simulink library "Motor_Lib"  (R2025a)
settings: Solver=ode45  StartTime=0.0  StopTime=10.0  RelTol=1e-3  EnableMultiTasking=on
libraries: fl_lib x44, ee_lib x1, $bdroot x1, sdl_lib x1
Description:
  | Copyright 2015-2025 The MathWorks, Inc.
settings Model: Creator=smiller  LastModifiedBy=smiller
settings SolverCC: AlgebraicLoopSolver=TrustRegion
settings DataIOCC: LimitDataPoints=on  SaveFormat=Array  ReturnWorkspaceOutputs=off
settings OptimizationCC: ReuseModelBlockBuffer=off  ExpressionDepthLimit=2147483647.0  LifeSpan=inf
settings DebuggingCC: UnderspecifiedInitializationDetection=Classic  MergeDetectMultiDrivingBlocksExec=none  SolverPrmCheckMsg=warning  UnconnectedInputMsg=warning  UnconnectedOutputMsg=warning  UnconnectedLineMsg=warning  AllowSymbolicDim=off  StateNameClashWarn=warning  PregeneratedLibrarySubsystemCodeDiagnostic=none  SFUnexpectedBacktrackingDiag=warning  SFNoUnconditionalDefaultTransitionDiag=warning  SFExecutionAtInitializationDiag=none  ArithmeticOperatorsInVariantConditions=warning
settings HardwareCC: ProdBitPerPointer=32.0  ProdBitPerSizeT=32.0  ProdBitPerPtrDiffT=32.0  ProdLargestAtomicFloat=None  ProdIntDivRoundTo=Undefined  ProdEndianess=Unspecified  ProdWordSize=32.0  ProdHWDeviceType=32-bit Generic
settings ModelReferenceCC: EnableRefExpFcnMdlSchedulingChecks=on  PropagateSignalLabelsOutOfModel=off
settings SFSimCC: SimUseLocalCustomCode=off  CustomCodeUndefinedFunction=UseInterfaceOnly
settings RTWCC: RTWUseLocalCustomCode=off  GPUComputeCapability=3.5  DLArmComputeVersion=19.05
settings CodeAppCC: StateflowObjectComments=on
settings GRTTargetCC: TargetLangStandard=C89/C90 (ANSI)
settings ConfigComp: CovMetricSettings=dw  CovSaveCumulativeToWorkspaceVar=on  CovSaveSingleToWorkspaceVar=on  CovExternalEMLEnable=off  CovSFcnEnable=off

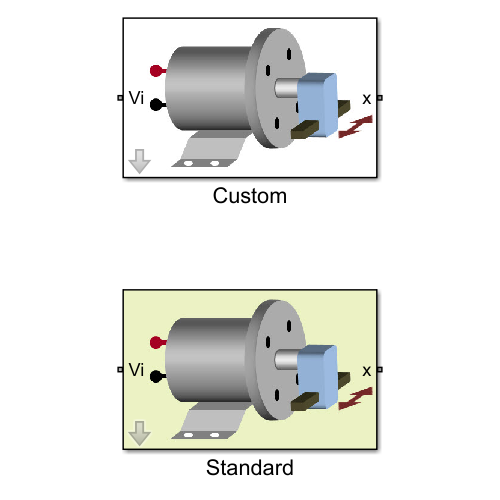
[thumbnail: Simulink's stored preview of the top-level diagram]
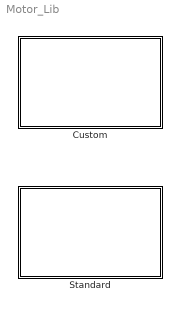
== system Motor_Lib ==
  Custom : Subsystem  mask(Servo and controller){G=0.5e-3/(pi/2), x_max=0.5, J=1e-4, lambda=0.01, R=10, L=2.5, Kt=0.04, R_controller=[10e3 10e3 10e3 100e3 50 100e3 10e3]}
      mask prompts: G "Spool travel per rotation (m)"; x_max "Spool travel limit (mm)"; J "Shaft inertia (kg m^2)"; lambda "Shaft damping (Nm/(rad/s))"; R "Winding resistance (ohms)"; L "Winding inductance (H)"; Kt "Torque constant (Nm/A)"; R_controller "[R1 R2 R3 R4 R5 R6 R7] (ohms)"
      mask help: Models a servomotor and controller using Simscape Foundation library components.
      mask DialogControl DescTextVar_copy Prompt: Controller resistance values
      mask Display: image('DC_Motor_Custom_IMAGE.jpg')
  Standard : Subsystem  mask(Servo and controller){G=0.5e-3/(pi/2), x_max=0.5, J=1e-4, lambda=0.01, R=10, L=2.5, Kt=0.04, R_controller=[10e3 10e3 10e3 100e3 50 100e3 10e3]}
      mask prompts: G "Spool travel per rotation (m)"; x_max "Spool travel limit (mm)"; J "Shaft inertia (kg m^2)"; lambda "Shaft damping (Nm/(rad/s))"; R "Winding resistance (ohms)"; L "Winding inductance (H)"; Kt "Torque constant (Nm/A)"; R_controller "[R1 R2 R3 R4 R5 R6 R7] (ohms)"
      mask help: Models a servomotor and controller using Simscape add-on library components.
      mask DialogControl DescTextVar_copy Prompt: Controller resistance values
      mask Display: image('DC_Motor_Standard_IMAGE.jpg')

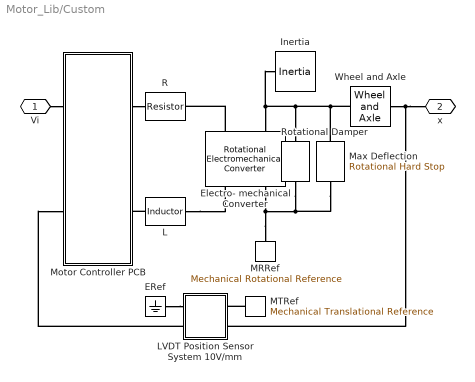
== system Motor_Lib/Custom ==
  ERef : fl_lib/Electrical/Electrical Elements/Electrical Reference
  Electro- mechanical Converter : fl_lib/Electrical/Electrical Elements/Rotational Electromechanical Converter  K=Kt V/(rad/s)  i_specify=off  i_priority=None  i=0 A  i_nominal_specify=off  i_nominal_value=1  i_nominal_unit=A  v_specify=off  v_priority=None  v=0 V  v_nominal_specify=off  v_nominal_value=1  v_nominal_unit=V  t_specify=off  t_priority=None  t=0 N*m  t_nominal_specify=off  t_nominal_value=1  t_nominal_unit=N*m  w_specify=off  w_priority=None  w=0 rad/s  w_nominal_specify=off  w_nominal_value=1  w_nominal_unit=rad/s
  Inertia : fl_lib/Mechanical/Rotational Elements/Inertia  inertia=J kg*m^2  num_ports=foundation.enum.numPorts2.one  w_specify=on  w_priority=High  w=0 rad/s  w_nominal_specify=off  w_nominal_value=1  w_nominal_unit=rad/s  t_specify=off  t_priority=None  t=0 N*m  t_nominal_specify=off  t_nominal_value=1  t_nominal_unit=N*m
  L : fl_lib/Electrical/Electrical Elements/Inductor  l=L H  r=0 Ohm  g=1e-09 1/Ohm  i_specify=off  i_priority=High  i=0 A  i_nominal_specify=off  i_nominal_value=1  i_nominal_unit=A  v_specify=off  v_priority=High  v=0 V  v_nominal_specify=off  v_nominal_value=1  v_nominal_unit=V  i_L_specify=on  i_L_priority=High  i_L=0 A  i_L_nominal_specify=off  i_L_nominal_value=1  i_L_nominal_unit=A
  LVDT Position Sensor System 10V/mm : Subsystem
  MRRef : fl_lib/Mechanical/Rotational Elements/Mechanical Rotational Reference
  MTRef : fl_lib/Mechanical/Translational Elements/Mechanical Translational Reference
  Max Deflection : fl_lib/Mechanical/Rotational Elements/Rotational Hard Stop  upper_bnd=x_max*1e-3/G rad  lower_bnd=-x_max*1e-3/G rad  model=3  stiff_up=1e+06 N*m/rad  stiff_low=1e+06 N*m/rad  D_up=0.05 N*m/(rad/s)  D_low=0.05 N*m/(rad/s)  transition=0.001 rad  coeff_rest=0.7  w_tol=0.1 rad/s  trq_tol=0.001 N*m  w_specify=off  w_priority=None  w=0 rad/s  w_nominal_specify=off  w_nominal_value=1  w_nominal_unit=rad/s  t_specify=off  t_priority=None  t=0 N*m  t_nominal_specify=off  t_nominal_value=1  t_nominal_unit=N*m  phi_specify=on  phi_priority=High  phi=0 rad  phi_nominal_specify=off  phi_nominal_value=1  phi_nominal_unit=rad  M_specify=off  M_priority=None  M=0
  Motor Controller PCB : Subsystem
  R : fl_lib/Electrical/Electrical Elements/Resistor  Tag=Factory Generic  R=R Ohm  i_specify=off  i_priority=High  i=0 A  i_nominal_specify=off  i_nominal_value=1  i_nominal_unit=A  v_specify=off  v_priority=High  v=0 V  v_nominal_specify=off  v_nominal_value=1  v_nominal_unit=V
  Rotational Damper : fl_lib/Mechanical/Rotational Elements/Rotational Damper  D=lambda N*m/(rad/s)  w_specify=off  w_priority=None  w=0 rad/s  w_nominal_specify=off  w_nominal_value=1  w_nominal_unit=rad/s  t_specify=off  t_priority=None  t=0 N*m  t_nominal_specify=off  t_nominal_value=1  t_nominal_unit=N*m
  Wheel and Axle : fl_lib/Mechanical/Mechanisms/Wheel and Axle  R=G m  or=1  t_specify=off  t_priority=High  t=0 N*m  t_nominal_specify=off  t_nominal_value=1  t_nominal_unit=N*m  f_specify=off  f_priority=High  f=0 N  f_nominal_specify=off  f_nominal_value=1  f_nominal_unit=N
  Vi : PMIOPort  Side=Left
  x : PMIOPort  Port=2  Side=Right
  connections:
  MTRef/LConn1 -- LVDT Position Sensor System 10V/mm/LConn1
  x/RConn1 -- Wheel and Axle/RConn1 -- LVDT Position Sensor System 10V/mm/LConn2
  L/RConn1 -- Electro- mechanical Converter/RConn1
  L/LConn1 -- Motor Controller PCB/RConn2
  Wheel and Axle/LConn1 -- Max Deflection/LConn1 -- Rotational Damper/LConn1 -- Electro- mechanical Converter/LConn2 -- Inertia/LConn1
  MRRef/LConn1 -- Electro- mechanical Converter/RConn2 -- Rotational Damper/RConn1 -- Max Deflection/RConn1
  Electro- mechanical Converter/LConn1 -- R/RConn1
  Motor Controller PCB/RConn1 -- R/LConn1
  Vi/RConn1 -- Motor Controller PCB/LConn1
  ERef/LConn1 -- LVDT Position Sensor System 10V/mm/RConn1
  LVDT Position Sensor System 10V/mm/RConn2 -- Motor Controller PCB/LConn2

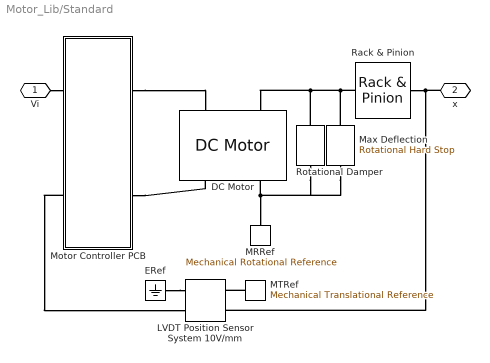
== system Motor_Lib/Standard ==
  DC Motor : ee_lib/Electromechanical/Brushed Motors/DC Motor  field_option=ee.enum.field_option.pm  Rf=100 Ohm  Lf=1 H  Laf=0.15 H  If0=0 A  parameterization=1  Ra=R Ohm  La=L H  emf_or_torque=1  Kv=Kt V/(rad/s)  Ki=6.876e-4 N*m/A  T_stall=2.4e-4 N*m  w_max=1.91e+4 rpm  w_rated=1.5e+4 rpm  P_rated=0.08 W  V_rated=1.5 V  lam_param=1  i_noload=0 A  V_i_noload=1.5 V  J=J kg*m^2  lam=0 N*m/(rad/s)  speed0=0 rpm  alpha=3.93e-3 1/K  Tmeas=25 degC  thermal_mass=100 J/K  initial_temperature=25 degC
  ERef : fl_lib/Electrical/Electrical Elements/Electrical Reference
  LVDT Position Sensor System 10V/mm : $bdroot/Custom/LVDT Position Sensor System 10V//mm  SystemSampleTime=-1  VariantActivationTime=update diagram  EmptyChoice=off  PassThrough=off  PassThroughVariantControl=(default)  EmptyChoiceVariantControl=(default)  AllowFlexibleInterface=on  Latency=0  AutoFrameSizeCalculation=off
  MRRef : fl_lib/Mechanical/Rotational Elements/Mechanical Rotational Reference
  MTRef : fl_lib/Mechanical/Translational Elements/Mechanical Translational Reference
  Max Deflection : fl_lib/Mechanical/Rotational Elements/Rotational Hard Stop  upper_bnd=x_max*1e-3/G rad  lower_bnd=-x_max*1e-3/G rad  model=3  stiff_up=1e+06 N*m/rad  stiff_low=1e+06 N*m/rad  D_up=0.05 N*m/(rad/s)  D_low=0.05 N*m/(rad/s)  transition=0.001 rad  coeff_rest=0.7  w_tol=0.1 rad/s  trq_tol=0.001 N*m  w_specify=off  w_priority=None  w=0 rad/s  w_nominal_specify=off  w_nominal_value=1  w_nominal_unit=rad/s  t_specify=off  t_priority=None  t=0 N*m  t_nominal_specify=off  t_nominal_value=1  t_nominal_unit=N*m  phi_specify=on  phi_priority=High  phi=0 rad  phi_nominal_specify=off  phi_nominal_value=1  phi_nominal_unit=rad  M_specify=off  M_priority=None  M=0
  Motor Controller PCB : Subsystem
  Rack & Pinion : sdl_lib/Gears/Rotational- Translational/Rack & Pinion  param=1  radius=G m  n_teeth=20  x_tooth=5 mm  rack_direction_sign=1  friction_model=1  efficiency=0.8  temperature_TLU=[ 280 300 320 ] K  efficiency_TLU=[ 0.95 0.9 0.85 ]  pwr_thr=0.001 W  mu_visc_P=0 N*m/(rad/s)  mu_visc_R=0 N/(m/s)  thermal_mass=50 J/K  temperature_specify=off  temperature_priority=High  temperature=300 K  temperature_nominal_specify=off  temperature_nominal_value=1  temperature_nominal_unit=K
      settings: InternalSimscapePortConfiguration="{\"Bottom\":[],\"Left\":[{\"id\":\"P\",\"label\":\"P\",\"type\":\"foundation.mechanical.rotational.rotational\"}],\"Right\":[{\"id\":\"R\",\"label\":\"R\",\"type\":\"foundation.mechanical.translational.translational\"}],\"Top\":[]}"
  Rotational Damper : fl_lib/Mechanical/Rotational Elements/Rotational Damper  D=lambda N*m/(rad/s)  w_specify=off  w_priority=None  w=0 rad/s  w_nominal_specify=off  w_nominal_value=1  w_nominal_unit=rad/s  t_specify=off  t_priority=None  t=0 N*m  t_nominal_specify=off  t_nominal_value=1  t_nominal_unit=N*m
  Vi : PMIOPort  Side=Left
  x : PMIOPort  Port=2  Side=Right
  connections:
  Vi/RConn1 -- Motor Controller PCB/LConn1
  Motor Controller PCB/RConn1 -- DC Motor/LConn1
  DC Motor/RConn2 -- Rotational Damper/RConn1 -- Max Deflection/RConn1 -- MRRef/LConn1
  Max Deflection/LConn1 -- Rotational Damper/LConn1 -- DC Motor/LConn2 -- Rack & Pinion/LConn1
  Motor Controller PCB/RConn2 -- DC Motor/RConn1
  ERef/LConn1 -- LVDT Position Sensor System 10V/mm/RConn1
  Motor Controller PCB/LConn2 -- LVDT Position Sensor System 10V/mm/RConn2
  MTRef/LConn1 -- LVDT Position Sensor System 10V/mm/LConn1
  x/RConn1 -- LVDT Position Sensor System 10V/mm/LConn2 -- Rack & Pinion/RConn1

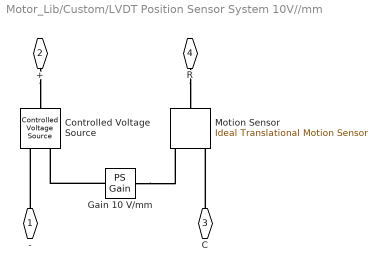
== system Motor_Lib/Custom/LVDT Position Sensor System 10V//mm ==
  Controlled Voltage Source : fl_lib/Electrical/Electrical Sources/Controlled Voltage Source
  Gain 10 V/mm : fl_lib/Physical Signals/Functions/PS Gain  gain=10 V/mm
  Motion Sensor : fl_lib/Mechanical/Mechanical Sensors/Ideal Translational Motion Sensor  reference=foundation.enum.MeasurementReference.difference  acceleration_port=false  velocity_port=true  position_port=true  offset=0 m
  - : PMIOPort  Side=Right
  + : PMIOPort  Port=2  Side=Right
  C : PMIOPort  Port=3  Side=Left
  R : PMIOPort  Port=4  Side=Left
  connections:
  Gain 10 V/mm/LConn1 -- Motion Sensor/RConn3
  C/RConn1 -- Motion Sensor/RConn1
  Gain 10 V/mm/RConn1 -- Controlled Voltage Source/RConn1
  R/RConn1 -- Motion Sensor/LConn1
  -/RConn1 -- Controlled Voltage Source/RConn2
  +/RConn1 -- Controlled Voltage Source/LConn1

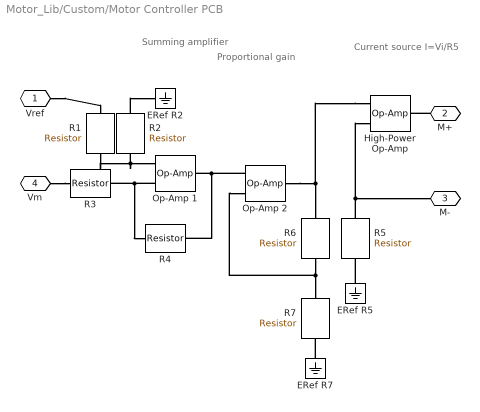
== system Motor_Lib/Custom/Motor Controller PCB ==
  note: Current source
      | I=Vi/R5
  note: Summing
      | amplifier
  note: Proportional gain
  ERef R2 : fl_lib/Electrical/Electrical Elements/Electrical Reference
  ERef R5 : fl_lib/Electrical/Electrical Elements/Electrical Reference
  ERef R7 : fl_lib/Electrical/Electrical Elements/Electrical Reference
  High-Power Op-Amp : fl_lib/Electrical/Electrical Elements/Op-Amp  outI_specify=off  outI_priority=High  outI=0 A  outI_nominal_specify=off  outI_nominal_value=1  outI_nominal_unit=A
  Op-Amp 1 : fl_lib/Electrical/Electrical Elements/Op-Amp  outI_specify=off  outI_priority=None  outI=0 A  outI_nominal_specify=off  outI_nominal_value=1  outI_nominal_unit=A
  Op-Amp 2 : fl_lib/Electrical/Electrical Elements/Op-Amp  outI_specify=off  outI_priority=None  outI=0 A  outI_nominal_specify=off  outI_nominal_value=1  outI_nominal_unit=A
  R1 : fl_lib/Electrical/Electrical Elements/Resistor  R=R_controller(1) Ohm  i_specify=off  i_priority=High  i=0 A  i_nominal_specify=off  i_nominal_value=1  i_nominal_unit=A  v_specify=off  v_priority=High  v=0 V  v_nominal_specify=off  v_nominal_value=1  v_nominal_unit=V
  R2 : fl_lib/Electrical/Electrical Elements/Resistor  R=R_controller(2) Ohm  i_specify=off  i_priority=None  i=0 A  i_nominal_specify=off  i_nominal_value=1  i_nominal_unit=A  v_specify=off  v_priority=None  v=0 V  v_nominal_specify=off  v_nominal_value=1  v_nominal_unit=V
  R3 : fl_lib/Electrical/Electrical Elements/Resistor  R=R_controller(3) Ohm  i_specify=off  i_priority=High  i=0 A  i_nominal_specify=off  i_nominal_value=1  i_nominal_unit=A  v_specify=off  v_priority=High  v=0 V  v_nominal_specify=off  v_nominal_value=1  v_nominal_unit=V
  R4 : fl_lib/Electrical/Electrical Elements/Resistor  R=R_controller(4) Ohm  i_specify=off  i_priority=None  i=0 A  i_nominal_specify=off  i_nominal_value=1  i_nominal_unit=A  v_specify=off  v_priority=None  v=0 V  v_nominal_specify=off  v_nominal_value=1  v_nominal_unit=V
  R5 : fl_lib/Electrical/Electrical Elements/Resistor  R=R_controller(5) Ohm  i_specify=off  i_priority=High  i=0 A  i_nominal_specify=off  i_nominal_value=1  i_nominal_unit=A  v_specify=off  v_priority=High  v=0 V  v_nominal_specify=off  v_nominal_value=1  v_nominal_unit=V
  R6 : fl_lib/Electrical/Electrical Elements/Resistor  R=R_controller(6) Ohm  i_specify=off  i_priority=None  i=0 A  i_nominal_specify=off  i_nominal_value=1  i_nominal_unit=A  v_specify=off  v_priority=None  v=0 V  v_nominal_specify=off  v_nominal_value=1  v_nominal_unit=V
  R7 : fl_lib/Electrical/Electrical Elements/Resistor  R=R_controller(7) Ohm  i_specify=off  i_priority=None  i=0 A  i_nominal_specify=off  i_nominal_value=1  i_nominal_unit=A  v_specify=off  v_priority=None  v=0 V  v_nominal_specify=off  v_nominal_value=1  v_nominal_unit=V
  Vref : PMIOPort  Side=Left
  M+ : PMIOPort  Port=2  Side=Right
  M- : PMIOPort  Port=3  Side=Right
  Vm : PMIOPort  Port=4  Side=Left
  connections:
  ERef R7/LConn1 -- R7/RConn1
  R2/RConn1 -- ERef R2/LConn1
  ERef R5/LConn1 -- R5/RConn1
  High-Power Op-Amp/LConn1 -- Op-Amp 2/RConn1 -- R6/LConn1
  R2/LConn1 -- Op-Amp 1/LConn1 -- R1/RConn1
  R3/RConn1 -- R4/LConn1 -- Op-Amp 1/LConn2
  Op-Amp 2/LConn1 -- Op-Amp 1/RConn1 -- R4/RConn1
  Op-Amp 2/LConn2 -- R7/LConn1 -- R6/RConn1
  Vref/RConn1 -- R1/LConn1
  M+/RConn1 -- High-Power Op-Amp/RConn1
  Vm/RConn1 -- R3/LConn1
  R5/LConn1 -- M-/RConn1 -- High-Power Op-Amp/LConn2

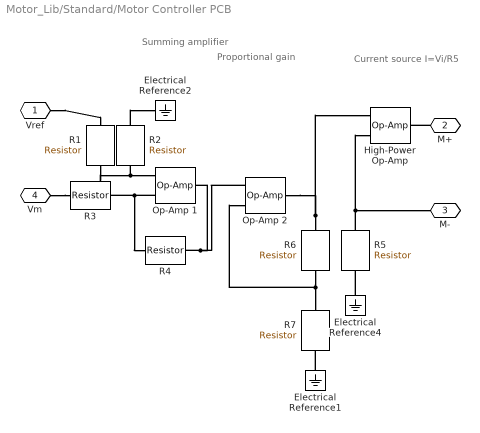
== system Motor_Lib/Standard/Motor Controller PCB ==
  note: Proportional gain
  note: Summing
      | amplifier
  note: Current source
      | I=Vi/R5
  Electrical Reference1 : fl_lib/Electrical/Electrical Elements/Electrical Reference
  Electrical Reference2 : fl_lib/Electrical/Electrical Elements/Electrical Reference
  Electrical Reference4 : fl_lib/Electrical/Electrical Elements/Electrical Reference
  High-Power Op-Amp : fl_lib/Electrical/Electrical Elements/Op-Amp  outI_specify=off  outI_priority=High  outI=0 A  outI_nominal_specify=off  outI_nominal_value=1  outI_nominal_unit=A
  Op-Amp 1 : fl_lib/Electrical/Electrical Elements/Op-Amp  outI_specify=off  outI_priority=None  outI=0 A  outI_nominal_specify=off  outI_nominal_value=1  outI_nominal_unit=A
  Op-Amp 2 : fl_lib/Electrical/Electrical Elements/Op-Amp  outI_specify=off  outI_priority=None  outI=0 A  outI_nominal_specify=off  outI_nominal_value=1  outI_nominal_unit=A
  R1 : fl_lib/Electrical/Electrical Elements/Resistor  R=R_controller(1) Ohm  i_specify=off  i_priority=High  i=0 A  i_nominal_specify=off  i_nominal_value=1  i_nominal_unit=A  v_specify=off  v_priority=High  v=0 V  v_nominal_specify=off  v_nominal_value=1  v_nominal_unit=V
  R2 : fl_lib/Electrical/Electrical Elements/Resistor  R=R_controller(2) Ohm  i_specify=off  i_priority=None  i=0 A  i_nominal_specify=off  i_nominal_value=1  i_nominal_unit=A  v_specify=off  v_priority=None  v=0 V  v_nominal_specify=off  v_nominal_value=1  v_nominal_unit=V
  R3 : fl_lib/Electrical/Electrical Elements/Resistor  R=R_controller(3) Ohm  i_specify=off  i_priority=High  i=0 A  i_nominal_specify=off  i_nominal_value=1  i_nominal_unit=A  v_specify=off  v_priority=High  v=0 V  v_nominal_specify=off  v_nominal_value=1  v_nominal_unit=V
  R4 : fl_lib/Electrical/Electrical Elements/Resistor  R=R_controller(4) Ohm  i_specify=off  i_priority=None  i=0 A  i_nominal_specify=off  i_nominal_value=1  i_nominal_unit=A  v_specify=off  v_priority=None  v=0 V  v_nominal_specify=off  v_nominal_value=1  v_nominal_unit=V
  R5 : fl_lib/Electrical/Electrical Elements/Resistor  R=R_controller(5) Ohm  i_specify=off  i_priority=High  i=0 A  i_nominal_specify=off  i_nominal_value=1  i_nominal_unit=A  v_specify=off  v_priority=High  v=0 V  v_nominal_specify=off  v_nominal_value=1  v_nominal_unit=V
  R6 : fl_lib/Electrical/Electrical Elements/Resistor  R=R_controller(6) Ohm  i_specify=off  i_priority=None  i=0 A  i_nominal_specify=off  i_nominal_value=1  i_nominal_unit=A  v_specify=off  v_priority=None  v=0 V  v_nominal_specify=off  v_nominal_value=1  v_nominal_unit=V
  R7 : fl_lib/Electrical/Electrical Elements/Resistor  R=R_controller(7) Ohm  i_specify=off  i_priority=None  i=0 A  i_nominal_specify=off  i_nominal_value=1  i_nominal_unit=A  v_specify=off  v_priority=None  v=0 V  v_nominal_specify=off  v_nominal_value=1  v_nominal_unit=V
  Vref : PMIOPort  Side=Left
  M+ : PMIOPort  Port=2  Side=Right
  M- : PMIOPort  Port=3  Side=Right
  Vm : PMIOPort  Port=4  Side=Left
  connections:
  Vm/RConn1 -- R3/LConn1
  M+/RConn1 -- High-Power Op-Amp/RConn1
  Vref/RConn1 -- R1/LConn1
  R6/RConn1 -- R7/LConn1 -- Op-Amp 2/LConn2
  R4/RConn1 -- Op-Amp 1/RConn1 -- Op-Amp 2/LConn1
  Op-Amp 1/LConn2 -- R4/LConn1 -- R3/RConn1
  R1/RConn1 -- Op-Amp 1/LConn1 -- R2/LConn1
  R6/LConn1 -- Op-Amp 2/RConn1 -- High-Power Op-Amp/LConn1
  Electrical Reference4/LConn1 -- R5/RConn1
  R2/RConn1 -- Electrical Reference2/LConn1
  Electrical Reference1/LConn1 -- R7/RConn1
  R5/LConn1 -- M-/RConn1 -- High-Power Op-Amp/LConn2
